simulink model "fix_Current_sync"  (R2025b)
settings: Solver=FixedStepAuto  StartTime=0.0  StopTime=20  FixedStep=0.001  RelTol=1e-3
values from neighbouring files (symbols this model uses):
  Dm = 1e-3    (= 0.001)    [motor_param.m]
  Ki_s = 0.041    [motor_param.m]
  Kp_s = 0.0014    [motor_param.m]
  Ld = 0.01    [motor_param.m]
  Lq = 0.02    [motor_param.m]
  p = 2    [motor_param.m]
  Phi = 0.1    [motor_param.m]
  Rs = 0.38    [motor_param.m]
libraries: fl_lib x50, nesl_utility x50, ee_lib x15, eeTransforms x10, slpidlib x5
(part 2 of 3)

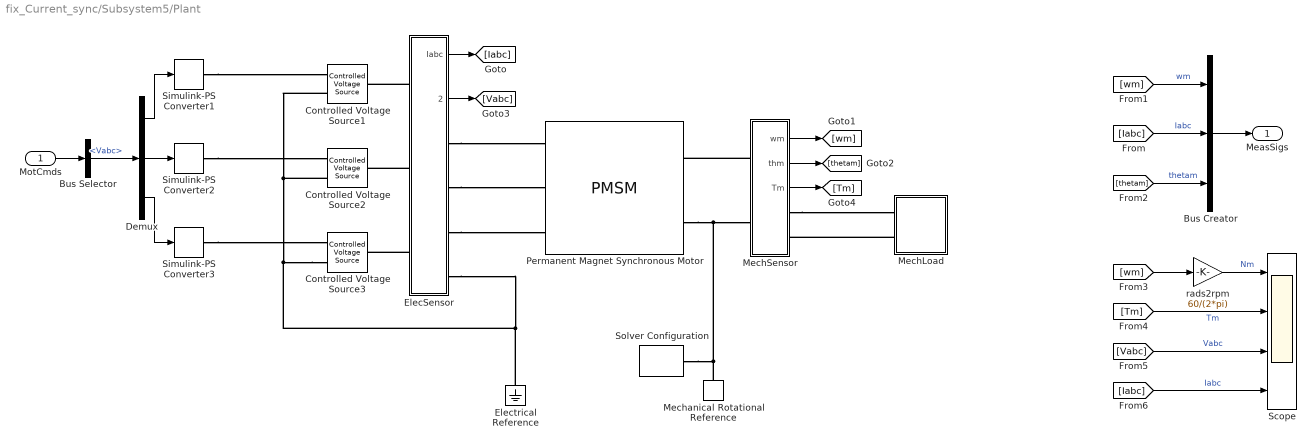
== system fix_Current_sync/Subsystem5/Plant ==
  MotCmds : Inport
  Bus Creator : BusCreator  Inputs=3
  Bus Selector : BusSelector  OutputSignals=Vabc
  Controlled Voltage Source1 : fl_lib/Electrical/Electrical Sources/Controlled Voltage Source
  Controlled Voltage Source2 : fl_lib/Electrical/Electrical Sources/Controlled Voltage Source
  Controlled Voltage Source3 : fl_lib/Electrical/Electrical Sources/Controlled Voltage Source
  Demux : Demux  Outputs=3
  ElecSensor : Subsystem
  Electrical Reference : fl_lib/Electrical/Electrical Elements/Electrical Reference
  MechLoad : Subsystem
  MechSensor : Subsystem
  Mechanical Rotational Reference : fl_lib/Mechanical/Rotational Elements/Mechanical Rotational Reference
  Permanent Magnet Synchronous Motor : ee_lib/Electromechanical/Permanent Magnet/PMSM  port_option=ee.enum.threePhasePort.expanded  winding_type=ee.enum.statorconnection.wye  machine_param=ee.enum.pmsm.parameterization.constant  nPolePairs=p  pmflux_param=1  pm_flux_linkage=Phi Wb  torque_constant=0.18 N*m/A  back_emf_constant=0.18 V/(rad/s)  stator_param=1  Ld=Ld H  Lq=Lq H  idVec=[-200, 0, 200] A  iqVec=[-200, 0, 200] A  LdMatrix=0.0002 * ones(3, 3) H  LqMatrix=0.0002 * ones(3, 3) H  PmMatrix=0.1 * ones(3, 3) Wb  ktMatrix=0.18 * ones(3, 3) N*m/A  keMatrix=0.18 * ones(3, 3) V/(rad/s)  L0=0 H  Ls=0.0002 H  Lm=-0.00002 H  Ms=0.00002 H  Rs=Rs Ohm  zero_sequence=ee.enum.park.zerosequence.exclude  axes_param=2  loss_param=ee.enum.ironloss.none  losses_oc=[0, 0, 0] W  losses_sc=[0, 0, 0] W  f_losses=60 Hz  Isc_losses=95 A  J=0 kg*m^2  lam=0 N*m/(rad/s)  i_d_specify=off  i_d_priority=None  i_d=0 A  i_d_nominal_specify=off  i_d_nominal_value=1  i_d_nominal_unit=A  i_q_specify=off  i_q_priority=None  i_q=0 A  i_q_nominal_specify=off  i_q_nominal_value=1  i_q_nominal_unit=A  torque_specify=off  torque_priority=None  torque=0 N*m  torque_nominal_specify=off  torque_nominal_value=1  torque_nominal_unit=N*m  angular_velocity_specify=on  angular_velocity_priority=High  angular_velocity=-100 rpm  angular_velocity_nominal_specify=off  angular_velocity_nominal_value=1  angular_velocity_nominal_unit=rpm  angular_position_specify=off  angular_position_priority=High  angular_position=2 rad  angular_position_nominal_specify=on  angular_position_nominal_value=10  angular_position_nominal_unit=deg  alpha=3.93e-3 1/K  alpha_flux=-0.001 1/K  Tmeas=298.15 K  stator_thermal_mass=100 J/K  rotor_thermal_mass=200 J/K  Rm_percent_rotor=90  Rd_percent_rotor=30  temperatureA_specify=off  temperatureA_priority=High  temperatureA=25 degC  temperatureA_nominal_specify=off  temperatureA_nominal_value=1  temperatureA_nominal_unit=degC  temperatureB_specify=off  temperatureB_priority=High  temperatureB=25 degC  temperatureB_nominal_specify=off  temperatureB_nominal_value=1  temperatureB_nominal_unit=degC  temperatureC_specify=off  temperatureC_priority=High  temperatureC=25 degC  temperatureC_nominal_specify=off  temperatureC_nominal_value=1  temperatureC_nominal_unit=degC  temperatureR_specify=off  temperatureR_priority=High  temperatureR=25 degC  temperatureR_nominal_specify=off  temperatureR_nominal_value=1  temperatureR_nominal_unit=degC
      settings: InternalSimscapePortConfiguration="{\"Bottom\":[],\"Left\":[{\"id\":\"a\",\"label\":\"a\",\"type\":\"foundation.electrical.electrical\"},{\"id\":\"b\",\"label\":\"b\",\"type\":\"foundation.electrical.electrical\"},{\"id\":\"c\",\"label\":\"c\",\"type\":\"foundation.electrical.electrical\"}],\"Right\":[{\"id\":\"R\",\"label\":\"R\",\"type\":\"foundation.mechanical.rotational.rotational\"},{\"id\":\"C\",\"label\":\"C\",\"type\":\"foundation.mechanical.rotational.rotational\"}],\"Top\":[]}"
  Scope : Scope  NumInputPorts=4
      settings: ActiveDisplayYMinimum=-2500.2768341970282  ActiveDisplayYMaximum=2500.1048598569782
  Simulink-PS Converter1 : nesl_utility/Simulink-PS Converter  PhysicalDomain=network_engine_domain  SubClassName=ps_input  LeftPortType=input  RightPortType=output  PseudoPeriodic=off  Frequencies=[]  NoiseDistribution=none  NoiseParameters=[]  Unit=1  AffineConversion=off  FilteringAndDerivatives=provide  SimscapeFilterOrder=1  InputFilterTimeConstant=1e-6  UdotUserProvided=0
  Simulink-PS Converter2 : nesl_utility/Simulink-PS Converter  PhysicalDomain=network_engine_domain  SubClassName=ps_input  LeftPortType=input  RightPortType=output  PseudoPeriodic=off  Frequencies=[]  NoiseDistribution=none  NoiseParameters=[]  Unit=1  AffineConversion=off  FilteringAndDerivatives=provide  SimscapeFilterOrder=1  InputFilterTimeConstant=1e-6  UdotUserProvided=0
  Simulink-PS Converter3 : nesl_utility/Simulink-PS Converter  PhysicalDomain=network_engine_domain  SubClassName=ps_input  LeftPortType=input  RightPortType=output  PseudoPeriodic=off  Frequencies=[]  NoiseDistribution=none  NoiseParameters=[]  Unit=1  AffineConversion=off  FilteringAndDerivatives=provide  SimscapeFilterOrder=1  InputFilterTimeConstant=1e-6  UdotUserProvided=0
  Solver Configuration : nesl_utility/Solver Configuration  PhysicalDomain=network_engine_domain  SubClassName=solver  LeftPortType=input  RightPortType=generic  Tones=[]  Harmonics=[]  SimulateNoise=off  Profile=off  UseLocalSampling=off  EnableSwitchedLinearOptims=on  FrequencyDomain=off  UseCCode=off  RelTol=0.001  AbsTol=1e-06  MinStep=1e-09  ToWorkspace=off  RevertToSquareIcSolve=off  NumHomotopyIterations=100  PhasorMode=off  PhasorModeNumHarmonics=1  ConsistencySolver=NEWTON_XTOL_AFTER_FTOL  IndexReductionMethod=DerivativeReplacement  DoDC=off  ResidualTolerance=1e-09  ConsistencyTolSource=GLOBAL  ConsistencyAbsTol=0.001  ConsistencyRelTol=0.001  ConsistencyTolFactor=0.001  UseLocalSolver=off  LocalSolverChoice=NE_BACKWARD_EULER_ADVANCER  ResolveIndetEquations=on  FunctionEvalNumThread=1  LocalSolverSampleTime=0.001  DoFixedCost=off  MaxNonlinIter=3  MaxModeIter=2  ComputeImpulses=off  ImpulseIterations=2  LinearAlgebra=Sparse  LinearAlgebraNumThread=0  EquationFormulation=NE_TIME_EF  DelaysMemoryBudget=1024  AutomaticFiltering=on  FilteringTimeConstant=0.001  PartitionStorageMethod=AS_NEEDED  PartitionMemoryBudget=1024  PartitionMethod=FAST  MultibodyUseLocalSolver=off  MultibodyLocalSolverChoice=ODE1  MultibodyLocalSolverSampleTime=0.001
  rads2rpm : Gain  Gain=60/(2*pi)
  MeasSigs : Outport  VectorParamsAs1DForOutWhenUnconnected=off
  wires:
  ElecSensor/1(Iabc) -> [Iabc]
  ElecSensor/2(Vabc) -> [Vabc]
  Demux/2 -> Simulink-PS Converter2/1
  Demux/1 -> Simulink-PS Converter1/1
  Demux/3 -> Simulink-PS Converter3/1
  MechSensor/1(wm) -> [wm]
  MechSensor/2(thm) -> [thetam]
  MechSensor/3(Tm) -> [Tm]
  [wm] -> Bus Creator/1  "wm"
  [Iabc] -> Bus Creator/2  "Iabc"
  [thetam] -> Bus Creator/3  "thetam"
  Bus Creator/1 -> MeasSigs/1
  MotCmds/1 -> Bus Selector/1
  Bus Selector/1 -> Demux/1  "<Vabc>"
  [wm] -> rads2rpm/1
  rads2rpm/1 -> Scope/1  "Nm"
  [Tm] -> Scope/2  "Tm"
  [Vabc] -> Scope/3  "Vabc"
  [Iabc] -> Scope/4  "Iabc"
  connections:
  Simulink-PS Converter2/RConn1 -- Controlled Voltage Source2/RConn1
  Simulink-PS Converter3/RConn1 -- Controlled Voltage Source3/RConn1
  ElecSensor/RConn3 -- Permanent Magnet Synchronous Motor/LConn3
  ElecSensor/LConn2 -- Controlled Voltage Source2/LConn1
  Controlled Voltage Source3/RConn2 -- Controlled Voltage Source1/RConn2 -- Controlled Voltage Source2/RConn2 -- ElecSensor/RConn4 -- Electrical Reference/LConn1
  ElecSensor/RConn2 -- Permanent Magnet Synchronous Motor/LConn2
  ElecSensor/RConn1 -- Permanent Magnet Synchronous Motor/LConn1
  ElecSensor/LConn3 -- Controlled Voltage Source3/LConn1
  ElecSensor/LConn1 -- Controlled Voltage Source1/LConn1
  Simulink-PS Converter1/RConn1 -- Controlled Voltage Source1/RConn1
  Permanent Magnet Synchronous Motor/RConn2 -- Solver Configuration/RConn1 -- Mechanical Rotational Reference/LConn1 -- MechSensor/LConn2
  MechSensor/RConn1 -- MechLoad/LConn1
  MechLoad/LConn2 -- MechSensor/RConn2
  MechSensor/LConn1 -- Permanent Magnet Synchronous Motor/RConn1

== system fix_Current_sync/Subsystem1/Controller/DriverPeripherals ==
  Vabc : Inport
  Break Algebraic Loop : Subsystem
  Bus Creator : BusCreator  Inputs=1
  MotCmds : Outport  VectorParamsAs1DForOutWhenUnconnected=off
  wires:
  Vabc/1 -> Break Algebraic Loop/1(In1)
  Bus Creator/1 -> MotCmds/1
  Break Algebraic Loop/1(Out1) -> Bus Creator/1  "Vabc"

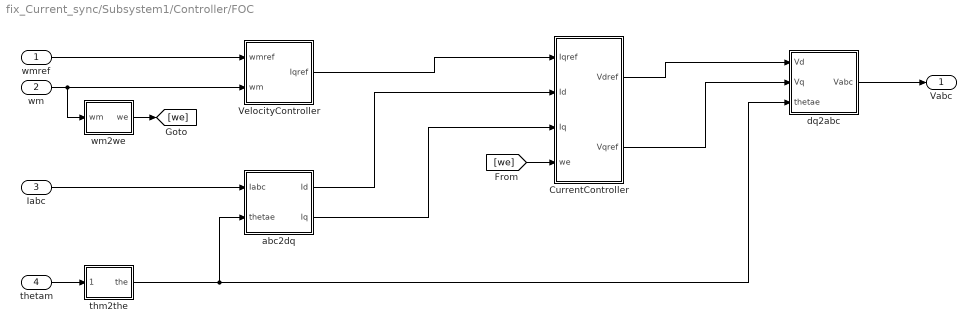
== system fix_Current_sync/Subsystem1/Controller/FOC ==
  wmref : Inport
  wm : Inport  Port=2
  Iabc : Inport  Port=3
  thetam : Inport  Port=4
  CurrentController : Subsystem
  VelocityController : Subsystem
  abc2dq : Subsystem
  dq2abc : Subsystem
  thm2the : Subsystem
  wm2we : Subsystem
  Vabc : Outport  VectorParamsAs1DForOutWhenUnconnected=off
  wires:
  abc2dq/2(Iq) -> CurrentController/3(Iq)
  wmref/1 -> VelocityController/1(wmref)
  abc2dq/1(Id) -> CurrentController/2(Id)
  Iabc/1 -> abc2dq/1(Iabc)
  CurrentController/1(Vdref) -> dq2abc/1(Vd)
  CurrentController/2(Vqref) -> dq2abc/2(Vq)
  [we] -> CurrentController/4(we)
  wm/1 -> VelocityController/2(wm), wm2we/1(wm)
  dq2abc/1(Vabc) -> Vabc/1
  VelocityController/1(Iqref) -> CurrentController/1(Iqref)
  thm2the/1(the) -> abc2dq/2(thetae), dq2abc/3(thetae)
  thetam/1 -> thm2the/1(thm)
  wm2we/1(we) -> [we]

== system fix_Current_sync/Subsystem1/Controller/SensorPeripherals ==
  MeasSigs : Inport
  Bus Selector : BusSelector  OutputSignals=wm,Iabc,thetam
  wm : Outport  VectorParamsAs1DForOutWhenUnconnected=off
  Iabc : Outport  Port=2  VectorParamsAs1DForOutWhenUnconnected=off
  thetam : Outport  Port=3  VectorParamsAs1DForOutWhenUnconnected=off
  wires:
  MeasSigs/1 -> Bus Selector/1
  Bus Selector/2 -> Iabc/1  "<Iabc>"
  Bus Selector/1 -> wm/1  "<wm>"
  Bus Selector/3 -> thetam/1  "<thetam>"

== system fix_Current_sync/Subsystem1/Controller/TestChannel ==
  TestSigs : Inport
  Bus Selector : BusSelector  OutputSignals=wmref
  wmref : Outport  VectorParamsAs1DForOutWhenUnconnected=off
  wires:
  TestSigs/1 -> Bus Selector/1
  Bus Selector/1 -> wmref/1  "<wmref>"

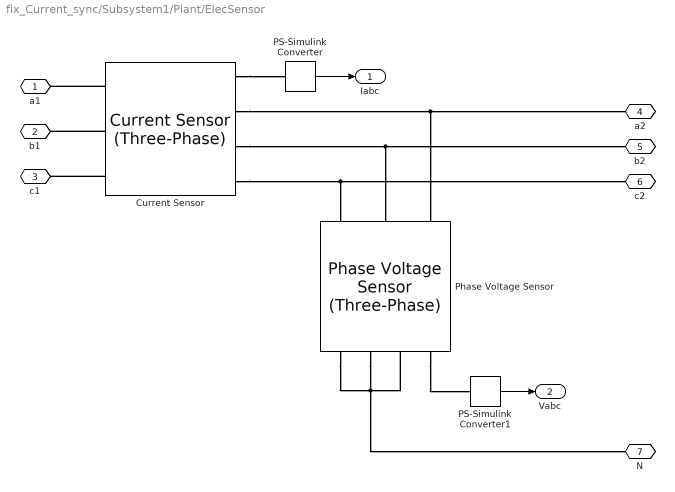
== system fix_Current_sync/Subsystem1/Plant/ElecSensor ==
  Current Sensor : ee_lib/Sensors & Transducers/Current Sensor (Three-Phase)
      settings: InternalSimscapePortConfiguration="{\"Bottom\":[],\"Left\":[{\"id\":\"a1\",\"label\":\"a1\",\"type\":\"foundation.electrical.electrical\"},{\"id\":\"b1\",\"label\":\"b1\",\"type\":\"foundation.electrical.electrical\"},{\"id\":\"c1\",\"label\":\"c1\",\"type\":\"foundation.electrical.electrical\"}],\"Right\":[{\"id\":\"I_output\",\"label\":\"I\",\"type\":\"output\"},{\"id\":\"a2\",\"label\":\"a2\",\"type\":\"foundation.electrical.electrical\"},{\"id\":\"b2\",\"label\":\"b2\",\"type\":\"foundation.electrical.electrical\"},{\"id\":\"c2\",\"label\":\"c2\",\"type\":\"foundation.electrical.electrical\"}],\"Top\":[]}"
  PS-Simulink Converter : nesl_utility/PS-Simulink Converter  PhysicalDomain=network_engine_domain  SubClassName=ps_output  LeftPortType=input  RightPortType=output  PseudoPeriodic=off  Frequencies=[]  VectorFormat=1-D array  Unit=1  AffineConversion=off
  PS-Simulink Converter1 : nesl_utility/PS-Simulink Converter  PhysicalDomain=network_engine_domain  SubClassName=ps_output  LeftPortType=input  RightPortType=output  PseudoPeriodic=off  Frequencies=[]  VectorFormat=1-D array  Unit=1  AffineConversion=off
  Phase Voltage Sensor : ee_lib/Sensors & Transducers/Phase Voltage Sensor (Three-Phase)
      settings: InternalSimscapePortConfiguration="{\"Bottom\":[],\"Left\":[{\"id\":\"a1\",\"label\":\"a1\",\"type\":\"foundation.electrical.electrical\"},{\"id\":\"b1\",\"label\":\"b1\",\"type\":\"foundation.electrical.electrical\"},{\"id\":\"c1\",\"label\":\"c1\",\"type\":\"foundation.electrical.electrical\"}],\"Right\":[{\"id\":\"V_output\",\"label\":\"V\",\"type\":\"output\"},{\"id\":\"a2\",\"label\":\"a2\",\"type\":\"foundation.electrical.electrical\"},{\"id\":\"b2\",\"label\":\"b2\",\"type\":\"foundation.electrical.electrical\"},{\"id\":\"c2\",\"label\":\"c2\",\"type\":\"foundation.electrical.electrical\"}],\"Top\":[]}"
  a1 : PMIOPort  Side=Left
  b1 : PMIOPort  Port=2  Side=Left
  c1 : PMIOPort  Port=3  Side=Left
  a2 : PMIOPort  Port=4  Side=Right
  b2 : PMIOPort  Port=5  Side=Right
  c2 : PMIOPort  Port=6  Side=Right
  N : PMIOPort  Port=7  Side=Right
  Iabc : Outport  VectorParamsAs1DForOutWhenUnconnected=off
  Vabc : Outport  Port=2  VectorParamsAs1DForOutWhenUnconnected=off
  wires:
  PS-Simulink Converter/1 -> Iabc/1
  PS-Simulink Converter1/1 -> Vabc/1
  connections:
  Current Sensor/LConn1 -- a1/RConn1
  Current Sensor/LConn2 -- b1/RConn1
  Current Sensor/LConn3 -- c1/RConn1
  Current Sensor/RConn1 -- PS-Simulink Converter/LConn1
  Phase Voltage Sensor/RConn1 -- PS-Simulink Converter1/LConn1
  Current Sensor/RConn2 -- a2/RConn1 -- Phase Voltage Sensor/LConn1
  Current Sensor/RConn3 -- b2/RConn1 -- Phase Voltage Sensor/LConn2
  Current Sensor/RConn4 -- c2/RConn1 -- Phase Voltage Sensor/LConn3
  Phase Voltage Sensor/RConn4 -- N/RConn1 -- Phase Voltage Sensor/RConn3 -- Phase Voltage Sensor/RConn2

== system fix_Current_sync/Subsystem1/Plant/MechLoad ==
  Ideal Torque Source : fl_lib/Mechanical/Mechanical Sources/Ideal Torque Source
  Inertia : fl_lib/Mechanical/Rotational Elements/Inertia  inertia=Jm kg*m^2  num_ports=foundation.enum.numPorts2.one  w_specify=on  w_priority=High  w=100 rpm  w_nominal_specify=off  w_nominal_value=1  w_nominal_unit=rad/s  t_specify=off  t_priority=None  t=0 N*m  t_nominal_specify=off  t_nominal_value=1  t_nominal_unit=N*m
  Rotational Damper : fl_lib/Mechanical/Rotational Elements/Rotational Damper  D=Dm N*m/(rad/s)  w_specify=off  w_priority=None  w=0 rad/s  w_nominal_specify=off  w_nominal_value=1  w_nominal_unit=rad/s  t_specify=off  t_priority=None  t=0 N*m  t_nominal_specify=off  t_nominal_value=1  t_nominal_unit=N*m
  Simulink-PS Converter4 : nesl_utility/Simulink-PS Converter  PhysicalDomain=network_engine_domain  SubClassName=ps_input  LeftPortType=input  RightPortType=output  PseudoPeriodic=off  Frequencies=[]  NoiseDistribution=none  NoiseParameters=[]  Unit=1  AffineConversion=off  FilteringAndDerivatives=provide  SimscapeFilterOrder=1  InputFilterTimeConstant=0.001  UdotUserProvided=0
  Step : Step  Time=0  After=0.2  SampleTime=0
  R : PMIOPort  Side=Left
  C : PMIOPort  Port=2  Side=Left
  wires:
  Step/1 -> Simulink-PS Converter4/1
  connections:
  Ideal Torque Source/RConn1 -- Simulink-PS Converter4/RConn1
  Rotational Damper/RConn1 -- Ideal Torque Source/RConn2 -- C/RConn1
  Rotational Damper/LConn1 -- Ideal Torque Source/LConn1 -- R/RConn1 -- Inertia/LConn1

== system fix_Current_sync/Subsystem1/Plant/MechSensor ==
  Ideal Rotational Motion Sensor : fl_lib/Mechanical/Mechanical Sensors/Ideal Rotational Motion Sensor  reference=foundation.enum.MeasurementReference.difference  acceleration_port=false  velocity_port=true  position_port=true  wrap_angle=simscape.enum.onoff.off  offset=0 rad
  Ideal Torque Sensor : fl_lib/Mechanical/Mechanical Sensors/Ideal Torque Sensor
  PS-Simulink Converter : nesl_utility/PS-Simulink Converter  PhysicalDomain=network_engine_domain  SubClassName=ps_output  LeftPortType=input  RightPortType=output  PseudoPeriodic=off  Frequencies=[]  VectorFormat=1-D array  Unit=1  AffineConversion=off
  PS-Simulink Converter1 : nesl_utility/PS-Simulink Converter  PhysicalDomain=network_engine_domain  SubClassName=ps_output  LeftPortType=input  RightPortType=output  PseudoPeriodic=off  Frequencies=[]  VectorFormat=1-D array  Unit=1  AffineConversion=off
  PS-Simulink Converter2 : nesl_utility/PS-Simulink Converter  PhysicalDomain=network_engine_domain  SubClassName=ps_output  LeftPortType=input  RightPortType=output  PseudoPeriodic=off  Frequencies=[]  VectorFormat=1-D array  Unit=1  AffineConversion=off
  R1 : PMIOPort  Side=Left
  C1 : PMIOPort  Port=2  Side=Left
  R2 : PMIOPort  Port=3  Side=Right
  C2 : PMIOPort  Port=4  Side=Right
  wm : Outport  VectorParamsAs1DForOutWhenUnconnected=off
  thm : Outport  Port=2  VectorParamsAs1DForOutWhenUnconnected=off
  Tm : Outport  Port=3  VectorParamsAs1DForOutWhenUnconnected=off
  wires:
  PS-Simulink Converter/1 -> thm/1
  PS-Simulink Converter1/1 -> Tm/1
  PS-Simulink Converter2/1 -> wm/1
  connections:
  Ideal Rotational Motion Sensor/RConn3 -- PS-Simulink Converter/LConn1
  Ideal Rotational Motion Sensor/RConn1 -- C2/RConn1 -- C1/RConn1
  Ideal Torque Sensor/LConn1 -- R1/RConn1
  Ideal Torque Sensor/RConn1 -- R2/RConn1 -- Ideal Rotational Motion Sensor/LConn1
  PS-Simulink Converter1/LConn1 -- Ideal Torque Sensor/RConn2
  Ideal Rotational Motion Sensor/RConn2 -- PS-Simulink Converter2/LConn1

== system fix_Current_sync/Subsystem2/Controller/DriverPeripherals ==
  Vabc : Inport
  Break Algebraic Loop : Subsystem
  Bus Creator : BusCreator  Inputs=1
  MotCmds : Outport  VectorParamsAs1DForOutWhenUnconnected=off
  wires:
  Vabc/1 -> Break Algebraic Loop/1(In1)
  Bus Creator/1 -> MotCmds/1
  Break Algebraic Loop/1(Out1) -> Bus Creator/1  "Vabc"

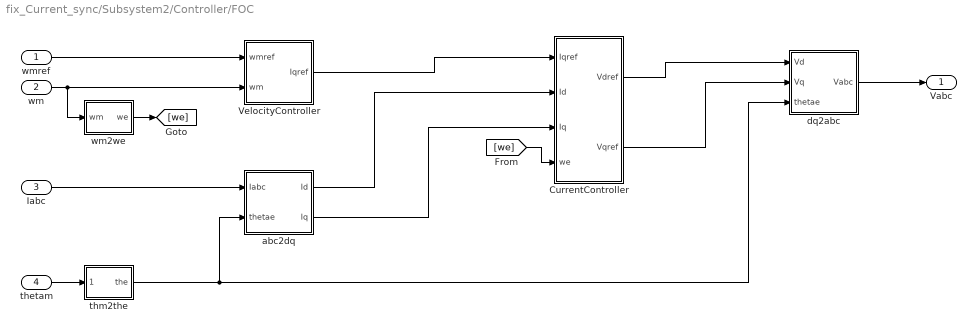
== system fix_Current_sync/Subsystem2/Controller/FOC ==
  wmref : Inport
  wm : Inport  Port=2
  Iabc : Inport  Port=3
  thetam : Inport  Port=4
  CurrentController : Subsystem
  VelocityController : Subsystem
  abc2dq : Subsystem
  dq2abc : Subsystem
  thm2the : Subsystem
  wm2we : Subsystem
  Vabc : Outport  VectorParamsAs1DForOutWhenUnconnected=off
  wires:
  abc2dq/2(Iq) -> CurrentController/3(Iq)
  wmref/1 -> VelocityController/1(wmref)
  abc2dq/1(Id) -> CurrentController/2(Id)
  Iabc/1 -> abc2dq/1(Iabc)
  CurrentController/1(Vdref) -> dq2abc/1(Vd)
  CurrentController/2(Vqref) -> dq2abc/2(Vq)
  [we] -> CurrentController/4(we)
  wm/1 -> VelocityController/2(wm), wm2we/1(wm)
  dq2abc/1(Vabc) -> Vabc/1
  VelocityController/1(Iqref) -> CurrentController/1(Iqref)
  thm2the/1(the) -> abc2dq/2(thetae), dq2abc/3(thetae)
  thetam/1 -> thm2the/1(thm)
  wm2we/1(we) -> [we]

== system fix_Current_sync/Subsystem2/Controller/SensorPeripherals ==
  MeasSigs : Inport
  Bus Selector : BusSelector  OutputSignals=wm,Iabc,thetam
  wm : Outport  VectorParamsAs1DForOutWhenUnconnected=off
  Iabc : Outport  Port=2  VectorParamsAs1DForOutWhenUnconnected=off
  thetam : Outport  Port=3  VectorParamsAs1DForOutWhenUnconnected=off
  wires:
  MeasSigs/1 -> Bus Selector/1
  Bus Selector/2 -> Iabc/1  "<Iabc>"
  Bus Selector/1 -> wm/1  "<wm>"
  Bus Selector/3 -> thetam/1  "<thetam>"

== system fix_Current_sync/Subsystem2/Controller/TestChannel ==
  TestSigs : Inport
  Bus Selector : BusSelector  OutputSignals=wmref
  wmref : Outport  VectorParamsAs1DForOutWhenUnconnected=off
  wires:
  TestSigs/1 -> Bus Selector/1
  Bus Selector/1 -> wmref/1  "<wmref>"

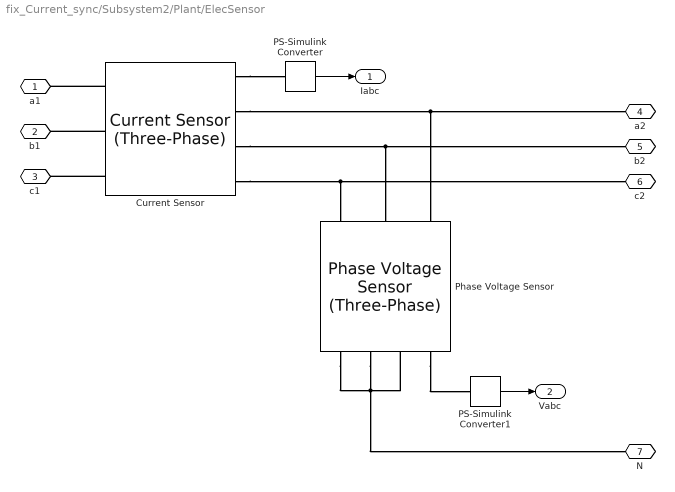
== system fix_Current_sync/Subsystem2/Plant/ElecSensor ==
  Current Sensor : ee_lib/Sensors & Transducers/Current Sensor (Three-Phase)
      settings: InternalSimscapePortConfiguration="{\"Bottom\":[],\"Left\":[{\"id\":\"a1\",\"label\":\"a1\",\"type\":\"foundation.electrical.electrical\"},{\"id\":\"b1\",\"label\":\"b1\",\"type\":\"foundation.electrical.electrical\"},{\"id\":\"c1\",\"label\":\"c1\",\"type\":\"foundation.electrical.electrical\"}],\"Right\":[{\"id\":\"I_output\",\"label\":\"I\",\"type\":\"output\"},{\"id\":\"a2\",\"label\":\"a2\",\"type\":\"foundation.electrical.electrical\"},{\"id\":\"b2\",\"label\":\"b2\",\"type\":\"foundation.electrical.electrical\"},{\"id\":\"c2\",\"label\":\"c2\",\"type\":\"foundation.electrical.electrical\"}],\"Top\":[]}"
  PS-Simulink Converter : nesl_utility/PS-Simulink Converter  PhysicalDomain=network_engine_domain  SubClassName=ps_output  LeftPortType=input  RightPortType=output  PseudoPeriodic=off  Frequencies=[]  VectorFormat=1-D array  Unit=1  AffineConversion=off
  PS-Simulink Converter1 : nesl_utility/PS-Simulink Converter  PhysicalDomain=network_engine_domain  SubClassName=ps_output  LeftPortType=input  RightPortType=output  PseudoPeriodic=off  Frequencies=[]  VectorFormat=1-D array  Unit=1  AffineConversion=off
  Phase Voltage Sensor : ee_lib/Sensors & Transducers/Phase Voltage Sensor (Three-Phase)
      settings: InternalSimscapePortConfiguration="{\"Bottom\":[],\"Left\":[{\"id\":\"a1\",\"label\":\"a1\",\"type\":\"foundation.electrical.electrical\"},{\"id\":\"b1\",\"label\":\"b1\",\"type\":\"foundation.electrical.electrical\"},{\"id\":\"c1\",\"label\":\"c1\",\"type\":\"foundation.electrical.electrical\"}],\"Right\":[{\"id\":\"V_output\",\"label\":\"V\",\"type\":\"output\"},{\"id\":\"a2\",\"label\":\"a2\",\"type\":\"foundation.electrical.electrical\"},{\"id\":\"b2\",\"label\":\"b2\",\"type\":\"foundation.electrical.electrical\"},{\"id\":\"c2\",\"label\":\"c2\",\"type\":\"foundation.electrical.electrical\"}],\"Top\":[]}"
  a1 : PMIOPort  Side=Left
  b1 : PMIOPort  Port=2  Side=Left
  c1 : PMIOPort  Port=3  Side=Left
  a2 : PMIOPort  Port=4  Side=Right
  b2 : PMIOPort  Port=5  Side=Right
  c2 : PMIOPort  Port=6  Side=Right
  N : PMIOPort  Port=7  Side=Right
  Iabc : Outport  VectorParamsAs1DForOutWhenUnconnected=off
  Vabc : Outport  Port=2  VectorParamsAs1DForOutWhenUnconnected=off
  wires:
  PS-Simulink Converter/1 -> Iabc/1
  PS-Simulink Converter1/1 -> Vabc/1
  connections:
  Current Sensor/LConn1 -- a1/RConn1
  Current Sensor/LConn2 -- b1/RConn1
  Current Sensor/LConn3 -- c1/RConn1
  Current Sensor/RConn1 -- PS-Simulink Converter/LConn1
  Phase Voltage Sensor/RConn1 -- PS-Simulink Converter1/LConn1
  Current Sensor/RConn2 -- a2/RConn1 -- Phase Voltage Sensor/LConn1
  Current Sensor/RConn3 -- b2/RConn1 -- Phase Voltage Sensor/LConn2
  Current Sensor/RConn4 -- c2/RConn1 -- Phase Voltage Sensor/LConn3
  Phase Voltage Sensor/RConn4 -- N/RConn1 -- Phase Voltage Sensor/RConn3 -- Phase Voltage Sensor/RConn2

== system fix_Current_sync/Subsystem2/Plant/MechLoad ==
  Ideal Torque Source : fl_lib/Mechanical/Mechanical Sources/Ideal Torque Source
  Inertia : fl_lib/Mechanical/Rotational Elements/Inertia  inertia=Jm kg*m^2  num_ports=foundation.enum.numPorts2.one  w_specify=on  w_priority=High  w=50 rpm  w_nominal_specify=off  w_nominal_value=1  w_nominal_unit=rad/s  t_specify=off  t_priority=None  t=0 N*m  t_nominal_specify=off  t_nominal_value=1  t_nominal_unit=N*m
  Rotational Damper : fl_lib/Mechanical/Rotational Elements/Rotational Damper  D=Dm N*m/(rad/s)  w_specify=off  w_priority=None  w=0 rad/s  w_nominal_specify=off  w_nominal_value=1  w_nominal_unit=rad/s  t_specify=off  t_priority=None  t=0 N*m  t_nominal_specify=off  t_nominal_value=1  t_nominal_unit=N*m
  Simulink-PS Converter4 : nesl_utility/Simulink-PS Converter  PhysicalDomain=network_engine_domain  SubClassName=ps_input  LeftPortType=input  RightPortType=output  PseudoPeriodic=off  Frequencies=[]  NoiseDistribution=none  NoiseParameters=[]  Unit=1  AffineConversion=off  FilteringAndDerivatives=provide  SimscapeFilterOrder=1  InputFilterTimeConstant=0.001  UdotUserProvided=0
  Step : Step  Time=0  After=0.5  SampleTime=0
  R : PMIOPort  Side=Left
  C : PMIOPort  Port=2  Side=Left
  wires:
  Step/1 -> Simulink-PS Converter4/1
  connections:
  Ideal Torque Source/RConn1 -- Simulink-PS Converter4/RConn1
  Rotational Damper/RConn1 -- Ideal Torque Source/RConn2 -- C/RConn1
  Rotational Damper/LConn1 -- Ideal Torque Source/LConn1 -- R/RConn1 -- Inertia/LConn1

== system fix_Current_sync/Subsystem2/Plant/MechSensor ==
  Ideal Rotational Motion Sensor : fl_lib/Mechanical/Mechanical Sensors/Ideal Rotational Motion Sensor  reference=foundation.enum.MeasurementReference.difference  acceleration_port=false  velocity_port=true  position_port=true  wrap_angle=simscape.enum.onoff.off  offset=0 rad
  Ideal Torque Sensor : fl_lib/Mechanical/Mechanical Sensors/Ideal Torque Sensor
  PS-Simulink Converter : nesl_utility/PS-Simulink Converter  PhysicalDomain=network_engine_domain  SubClassName=ps_output  LeftPortType=input  RightPortType=output  PseudoPeriodic=off  Frequencies=[]  VectorFormat=1-D array  Unit=1  AffineConversion=off
  PS-Simulink Converter1 : nesl_utility/PS-Simulink Converter  PhysicalDomain=network_engine_domain  SubClassName=ps_output  LeftPortType=input  RightPortType=output  PseudoPeriodic=off  Frequencies=[]  VectorFormat=1-D array  Unit=1  AffineConversion=off
  PS-Simulink Converter2 : nesl_utility/PS-Simulink Converter  PhysicalDomain=network_engine_domain  SubClassName=ps_output  LeftPortType=input  RightPortType=output  PseudoPeriodic=off  Frequencies=[]  VectorFormat=1-D array  Unit=1  AffineConversion=off
  R1 : PMIOPort  Side=Left
  C1 : PMIOPort  Port=2  Side=Left
  R2 : PMIOPort  Port=3  Side=Right
  C2 : PMIOPort  Port=4  Side=Right
  wm : Outport  VectorParamsAs1DForOutWhenUnconnected=off
  thm : Outport  Port=2  VectorParamsAs1DForOutWhenUnconnected=off
  Tm : Outport  Port=3  VectorParamsAs1DForOutWhenUnconnected=off
  wires:
  PS-Simulink Converter/1 -> thm/1
  PS-Simulink Converter1/1 -> Tm/1
  PS-Simulink Converter2/1 -> wm/1
  connections:
  Ideal Rotational Motion Sensor/RConn3 -- PS-Simulink Converter/LConn1
  Ideal Rotational Motion Sensor/RConn1 -- C2/RConn1 -- C1/RConn1
  Ideal Torque Sensor/LConn1 -- R1/RConn1
  Ideal Torque Sensor/RConn1 -- R2/RConn1 -- Ideal Rotational Motion Sensor/LConn1
  PS-Simulink Converter1/LConn1 -- Ideal Torque Sensor/RConn2
  Ideal Rotational Motion Sensor/RConn2 -- PS-Simulink Converter2/LConn1

== system fix_Current_sync/Subsystem3/Controller/DriverPeripherals ==
  Vabc : Inport
  Break Algebraic Loop : Subsystem
  Bus Creator : BusCreator  Inputs=1
  MotCmds : Outport  VectorParamsAs1DForOutWhenUnconnected=off
  wires:
  Vabc/1 -> Break Algebraic Loop/1(In1)
  Bus Creator/1 -> MotCmds/1
  Break Algebraic Loop/1(Out1) -> Bus Creator/1  "Vabc"

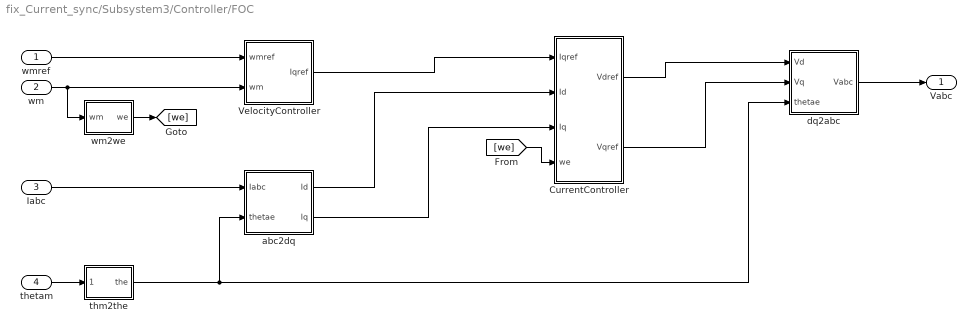
== system fix_Current_sync/Subsystem3/Controller/FOC ==
  wmref : Inport
  wm : Inport  Port=2
  Iabc : Inport  Port=3
  thetam : Inport  Port=4
  CurrentController : Subsystem
  VelocityController : Subsystem
  abc2dq : Subsystem
  dq2abc : Subsystem
  thm2the : Subsystem
  wm2we : Subsystem
  Vabc : Outport  VectorParamsAs1DForOutWhenUnconnected=off
  wires:
  abc2dq/2(Iq) -> CurrentController/3(Iq)
  wmref/1 -> VelocityController/1(wmref)
  abc2dq/1(Id) -> CurrentController/2(Id)
  Iabc/1 -> abc2dq/1(Iabc)
  CurrentController/1(Vdref) -> dq2abc/1(Vd)
  CurrentController/2(Vqref) -> dq2abc/2(Vq)
  [we] -> CurrentController/4(we)
  wm/1 -> VelocityController/2(wm), wm2we/1(wm)
  dq2abc/1(Vabc) -> Vabc/1
  VelocityController/1(Iqref) -> CurrentController/1(Iqref)
  thm2the/1(the) -> abc2dq/2(thetae), dq2abc/3(thetae)
  thetam/1 -> thm2the/1(thm)
  wm2we/1(we) -> [we]

== system fix_Current_sync/Subsystem3/Controller/SensorPeripherals ==
  MeasSigs : Inport
  Bus Selector : BusSelector  OutputSignals=wm,Iabc,thetam
  wm : Outport  VectorParamsAs1DForOutWhenUnconnected=off
  Iabc : Outport  Port=2  VectorParamsAs1DForOutWhenUnconnected=off
  thetam : Outport  Port=3  VectorParamsAs1DForOutWhenUnconnected=off
  wires:
  MeasSigs/1 -> Bus Selector/1
  Bus Selector/2 -> Iabc/1  "<Iabc>"
  Bus Selector/1 -> wm/1  "<wm>"
  Bus Selector/3 -> thetam/1  "<thetam>"

== system fix_Current_sync/Subsystem3/Controller/TestChannel ==
  TestSigs : Inport
  Bus Selector : BusSelector  OutputSignals=wmref
  wmref : Outport  VectorParamsAs1DForOutWhenUnconnected=off
  wires:
  TestSigs/1 -> Bus Selector/1
  Bus Selector/1 -> wmref/1  "<wmref>"

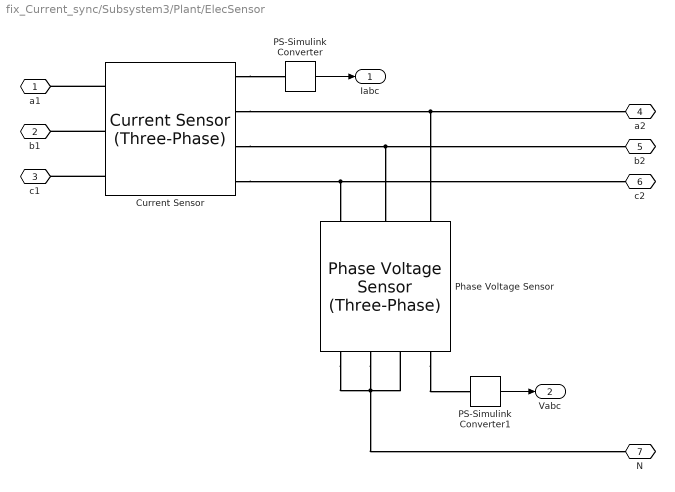
== system fix_Current_sync/Subsystem3/Plant/ElecSensor ==
  Current Sensor : ee_lib/Sensors & Transducers/Current Sensor (Three-Phase)
      settings: InternalSimscapePortConfiguration="{\"Bottom\":[],\"Left\":[{\"id\":\"a1\",\"label\":\"a1\",\"type\":\"foundation.electrical.electrical\"},{\"id\":\"b1\",\"label\":\"b1\",\"type\":\"foundation.electrical.electrical\"},{\"id\":\"c1\",\"label\":\"c1\",\"type\":\"foundation.electrical.electrical\"}],\"Right\":[{\"id\":\"I_output\",\"label\":\"I\",\"type\":\"output\"},{\"id\":\"a2\",\"label\":\"a2\",\"type\":\"foundation.electrical.electrical\"},{\"id\":\"b2\",\"label\":\"b2\",\"type\":\"foundation.electrical.electrical\"},{\"id\":\"c2\",\"label\":\"c2\",\"type\":\"foundation.electrical.electrical\"}],\"Top\":[]}"
  PS-Simulink Converter : nesl_utility/PS-Simulink Converter  PhysicalDomain=network_engine_domain  SubClassName=ps_output  LeftPortType=input  RightPortType=output  PseudoPeriodic=off  Frequencies=[]  VectorFormat=1-D array  Unit=1  AffineConversion=off
  PS-Simulink Converter1 : nesl_utility/PS-Simulink Converter  PhysicalDomain=network_engine_domain  SubClassName=ps_output  LeftPortType=input  RightPortType=output  PseudoPeriodic=off  Frequencies=[]  VectorFormat=1-D array  Unit=1  AffineConversion=off
  Phase Voltage Sensor : ee_lib/Sensors & Transducers/Phase Voltage Sensor (Three-Phase)
      settings: InternalSimscapePortConfiguration="{\"Bottom\":[],\"Left\":[{\"id\":\"a1\",\"label\":\"a1\",\"type\":\"foundation.electrical.electrical\"},{\"id\":\"b1\",\"label\":\"b1\",\"type\":\"foundation.electrical.electrical\"},{\"id\":\"c1\",\"label\":\"c1\",\"type\":\"foundation.electrical.electrical\"}],\"Right\":[{\"id\":\"V_output\",\"label\":\"V\",\"type\":\"output\"},{\"id\":\"a2\",\"label\":\"a2\",\"type\":\"foundation.electrical.electrical\"},{\"id\":\"b2\",\"label\":\"b2\",\"type\":\"foundation.electrical.electrical\"},{\"id\":\"c2\",\"label\":\"c2\",\"type\":\"foundation.electrical.electrical\"}],\"Top\":[]}"
  a1 : PMIOPort  Side=Left
  b1 : PMIOPort  Port=2  Side=Left
  c1 : PMIOPort  Port=3  Side=Left
  a2 : PMIOPort  Port=4  Side=Right
  b2 : PMIOPort  Port=5  Side=Right
  c2 : PMIOPort  Port=6  Side=Right
  N : PMIOPort  Port=7  Side=Right
  Iabc : Outport  VectorParamsAs1DForOutWhenUnconnected=off
  Vabc : Outport  Port=2  VectorParamsAs1DForOutWhenUnconnected=off
  wires:
  PS-Simulink Converter/1 -> Iabc/1
  PS-Simulink Converter1/1 -> Vabc/1
  connections:
  Current Sensor/LConn1 -- a1/RConn1
  Current Sensor/LConn2 -- b1/RConn1
  Current Sensor/LConn3 -- c1/RConn1
  Current Sensor/RConn1 -- PS-Simulink Converter/LConn1
  Phase Voltage Sensor/RConn1 -- PS-Simulink Converter1/LConn1
  Current Sensor/RConn2 -- a2/RConn1 -- Phase Voltage Sensor/LConn1
  Current Sensor/RConn3 -- b2/RConn1 -- Phase Voltage Sensor/LConn2
  Current Sensor/RConn4 -- c2/RConn1 -- Phase Voltage Sensor/LConn3
  Phase Voltage Sensor/RConn4 -- N/RConn1 -- Phase Voltage Sensor/RConn3 -- Phase Voltage Sensor/RConn2

== system fix_Current_sync/Subsystem3/Plant/MechLoad ==
  Ideal Torque Source : fl_lib/Mechanical/Mechanical Sources/Ideal Torque Source
  Inertia : fl_lib/Mechanical/Rotational Elements/Inertia  inertia=Jm kg*m^2  num_ports=foundation.enum.numPorts2.one  w_specify=on  w_priority=High  w=0 rpm  w_nominal_specify=off  w_nominal_value=1  w_nominal_unit=rad/s  t_specify=off  t_priority=None  t=0 N*m  t_nominal_specify=off  t_nominal_value=1  t_nominal_unit=N*m
  Rotational Damper : fl_lib/Mechanical/Rotational Elements/Rotational Damper  D=Dm N*m/(rad/s)  w_specify=off  w_priority=None  w=0 rad/s  w_nominal_specify=off  w_nominal_value=1  w_nominal_unit=rad/s  t_specify=off  t_priority=None  t=0 N*m  t_nominal_specify=off  t_nominal_value=1  t_nominal_unit=N*m
  Simulink-PS Converter4 : nesl_utility/Simulink-PS Converter  PhysicalDomain=network_engine_domain  SubClassName=ps_input  LeftPortType=input  RightPortType=output  PseudoPeriodic=off  Frequencies=[]  NoiseDistribution=none  NoiseParameters=[]  Unit=1  AffineConversion=off  FilteringAndDerivatives=provide  SimscapeFilterOrder=1  InputFilterTimeConstant=0.001  UdotUserProvided=0
  Step : Step  Time=0  After=-0.2  SampleTime=0
  R : PMIOPort  Side=Left
  C : PMIOPort  Port=2  Side=Left
  wires:
  Step/1 -> Simulink-PS Converter4/1
  connections:
  Ideal Torque Source/RConn1 -- Simulink-PS Converter4/RConn1
  Rotational Damper/RConn1 -- Ideal Torque Source/RConn2 -- C/RConn1
  Rotational Damper/LConn1 -- Ideal Torque Source/LConn1 -- R/RConn1 -- Inertia/LConn1

== system fix_Current_sync/Subsystem3/Plant/MechSensor ==
  Ideal Rotational Motion Sensor : fl_lib/Mechanical/Mechanical Sensors/Ideal Rotational Motion Sensor  reference=foundation.enum.MeasurementReference.difference  acceleration_port=false  velocity_port=true  position_port=true  wrap_angle=simscape.enum.onoff.off  offset=0 rad
  Ideal Torque Sensor : fl_lib/Mechanical/Mechanical Sensors/Ideal Torque Sensor
  PS-Simulink Converter : nesl_utility/PS-Simulink Converter  PhysicalDomain=network_engine_domain  SubClassName=ps_output  LeftPortType=input  RightPortType=output  PseudoPeriodic=off  Frequencies=[]  VectorFormat=1-D array  Unit=1  AffineConversion=off
  PS-Simulink Converter1 : nesl_utility/PS-Simulink Converter  PhysicalDomain=network_engine_domain  SubClassName=ps_output  LeftPortType=input  RightPortType=output  PseudoPeriodic=off  Frequencies=[]  VectorFormat=1-D array  Unit=1  AffineConversion=off
  PS-Simulink Converter2 : nesl_utility/PS-Simulink Converter  PhysicalDomain=network_engine_domain  SubClassName=ps_output  LeftPortType=input  RightPortType=output  PseudoPeriodic=off  Frequencies=[]  VectorFormat=1-D array  Unit=1  AffineConversion=off
  R1 : PMIOPort  Side=Left
  C1 : PMIOPort  Port=2  Side=Left
  R2 : PMIOPort  Port=3  Side=Right
  C2 : PMIOPort  Port=4  Side=Right
  wm : Outport  VectorParamsAs1DForOutWhenUnconnected=off
  thm : Outport  Port=2  VectorParamsAs1DForOutWhenUnconnected=off
  Tm : Outport  Port=3  VectorParamsAs1DForOutWhenUnconnected=off
  wires:
  PS-Simulink Converter/1 -> thm/1
  PS-Simulink Converter1/1 -> Tm/1
  PS-Simulink Converter2/1 -> wm/1
  connections:
  Ideal Rotational Motion Sensor/RConn3 -- PS-Simulink Converter/LConn1
  Ideal Rotational Motion Sensor/RConn1 -- C2/RConn1 -- C1/RConn1
  Ideal Torque Sensor/LConn1 -- R1/RConn1
  Ideal Torque Sensor/RConn1 -- R2/RConn1 -- Ideal Rotational Motion Sensor/LConn1
  PS-Simulink Converter1/LConn1 -- Ideal Torque Sensor/RConn2
  Ideal Rotational Motion Sensor/RConn2 -- PS-Simulink Converter2/LConn1

== system fix_Current_sync/Subsystem4/Controller/DriverPeripherals ==
  Vabc : Inport
  Break Algebraic Loop : Subsystem
  Bus Creator : BusCreator  Inputs=1
  MotCmds : Outport  VectorParamsAs1DForOutWhenUnconnected=off
  wires:
  Vabc/1 -> Break Algebraic Loop/1(In1)
  Bus Creator/1 -> MotCmds/1
  Break Algebraic Loop/1(Out1) -> Bus Creator/1  "Vabc"

== system fix_Current_sync/Subsystem4/Controller/FOC ==
  wmref : Inport
  wm : Inport  Port=2
  Iabc : Inport  Port=3
  thetam : Inport  Port=4
  CurrentController : Subsystem
  VelocityController : Subsystem
  abc2dq : Subsystem
  dq2abc : Subsystem
  thm2the : Subsystem
  wm2we : Subsystem
  Vabc : Outport  VectorParamsAs1DForOutWhenUnconnected=off
  wires:
  abc2dq/2(Iq) -> CurrentController/3(Iq)
  wmref/1 -> VelocityController/1(wmref)
  abc2dq/1(Id) -> CurrentController/2(Id)
  Iabc/1 -> abc2dq/1(Iabc)
  CurrentController/1(Vdref) -> dq2abc/1(Vd)
  CurrentController/2(Vqref) -> dq2abc/2(Vq)
  [we] -> CurrentController/4(we)
  wm/1 -> VelocityController/2(wm), wm2we/1(wm)
  dq2abc/1(Vabc) -> Vabc/1
  VelocityController/1(Iqref) -> CurrentController/1(Iqref)
  thm2the/1(the) -> abc2dq/2(thetae), dq2abc/3(thetae)
  thetam/1 -> thm2the/1(thm)
  wm2we/1(we) -> [we]

== system fix_Current_sync/Subsystem4/Controller/SensorPeripherals ==
  MeasSigs : Inport
  Bus Selector : BusSelector  OutputSignals=wm,Iabc,thetam
  wm : Outport  VectorParamsAs1DForOutWhenUnconnected=off
  Iabc : Outport  Port=2  VectorParamsAs1DForOutWhenUnconnected=off
  thetam : Outport  Port=3  VectorParamsAs1DForOutWhenUnconnected=off
  wires:
  MeasSigs/1 -> Bus Selector/1
  Bus Selector/2 -> Iabc/1  "<Iabc>"
  Bus Selector/1 -> wm/1  "<wm>"
  Bus Selector/3 -> thetam/1  "<thetam>"

== system fix_Current_sync/Subsystem4/Controller/TestChannel ==
  TestSigs : Inport
  Bus Selector : BusSelector  OutputSignals=wmref
  wmref : Outport  VectorParamsAs1DForOutWhenUnconnected=off
  wires:
  TestSigs/1 -> Bus Selector/1
  Bus Selector/1 -> wmref/1  "<wmref>"

== system fix_Current_sync/Subsystem4/Plant/ElecSensor ==
  Current Sensor : ee_lib/Sensors & Transducers/Current Sensor (Three-Phase)
      settings: InternalSimscapePortConfiguration="{\"Bottom\":[],\"Left\":[{\"id\":\"a1\",\"label\":\"a1\",\"type\":\"foundation.electrical.electrical\"},{\"id\":\"b1\",\"label\":\"b1\",\"type\":\"foundation.electrical.electrical\"},{\"id\":\"c1\",\"label\":\"c1\",\"type\":\"foundation.electrical.electrical\"}],\"Right\":[{\"id\":\"I_output\",\"label\":\"I\",\"type\":\"output\"},{\"id\":\"a2\",\"label\":\"a2\",\"type\":\"foundation.electrical.electrical\"},{\"id\":\"b2\",\"label\":\"b2\",\"type\":\"foundation.electrical.electrical\"},{\"id\":\"c2\",\"label\":\"c2\",\"type\":\"foundation.electrical.electrical\"}],\"Top\":[]}"
  PS-Simulink Converter : nesl_utility/PS-Simulink Converter  PhysicalDomain=network_engine_domain  SubClassName=ps_output  LeftPortType=input  RightPortType=output  PseudoPeriodic=off  Frequencies=[]  VectorFormat=1-D array  Unit=1  AffineConversion=off
  PS-Simulink Converter1 : nesl_utility/PS-Simulink Converter  PhysicalDomain=network_engine_domain  SubClassName=ps_output  LeftPortType=input  RightPortType=output  PseudoPeriodic=off  Frequencies=[]  VectorFormat=1-D array  Unit=1  AffineConversion=off
  Phase Voltage Sensor : ee_lib/Sensors & Transducers/Phase Voltage Sensor (Three-Phase)
      settings: InternalSimscapePortConfiguration="{\"Bottom\":[],\"Left\":[{\"id\":\"a1\",\"label\":\"a1\",\"type\":\"foundation.electrical.electrical\"},{\"id\":\"b1\",\"label\":\"b1\",\"type\":\"foundation.electrical.electrical\"},{\"id\":\"c1\",\"label\":\"c1\",\"type\":\"foundation.electrical.electrical\"}],\"Right\":[{\"id\":\"V_output\",\"label\":\"V\",\"type\":\"output\"},{\"id\":\"a2\",\"label\":\"a2\",\"type\":\"foundation.electrical.electrical\"},{\"id\":\"b2\",\"label\":\"b2\",\"type\":\"foundation.electrical.electrical\"},{\"id\":\"c2\",\"label\":\"c2\",\"type\":\"foundation.electrical.electrical\"}],\"Top\":[]}"
  a1 : PMIOPort  Side=Left
  b1 : PMIOPort  Port=2  Side=Left
  c1 : PMIOPort  Port=3  Side=Left
  a2 : PMIOPort  Port=4  Side=Right
  b2 : PMIOPort  Port=5  Side=Right
  c2 : PMIOPort  Port=6  Side=Right
  N : PMIOPort  Port=7  Side=Right
  Iabc : Outport  VectorParamsAs1DForOutWhenUnconnected=off
  Vabc : Outport  Port=2  VectorParamsAs1DForOutWhenUnconnected=off
  wires:
  PS-Simulink Converter/1 -> Iabc/1
  PS-Simulink Converter1/1 -> Vabc/1
  connections:
  Current Sensor/LConn1 -- a1/RConn1
  Current Sensor/LConn2 -- b1/RConn1
  Current Sensor/LConn3 -- c1/RConn1
  Current Sensor/RConn1 -- PS-Simulink Converter/LConn1
  Phase Voltage Sensor/RConn1 -- PS-Simulink Converter1/LConn1
  Current Sensor/RConn2 -- a2/RConn1 -- Phase Voltage Sensor/LConn1
  Current Sensor/RConn3 -- b2/RConn1 -- Phase Voltage Sensor/LConn2
  Current Sensor/RConn4 -- c2/RConn1 -- Phase Voltage Sensor/LConn3
  Phase Voltage Sensor/RConn4 -- N/RConn1 -- Phase Voltage Sensor/RConn3 -- Phase Voltage Sensor/RConn2

== system fix_Current_sync/Subsystem4/Plant/MechLoad ==
  Ideal Torque Source : fl_lib/Mechanical/Mechanical Sources/Ideal Torque Source
  Inertia : fl_lib/Mechanical/Rotational Elements/Inertia  inertia=Jm kg*m^2  num_ports=foundation.enum.numPorts2.one  w_specify=on  w_priority=High  w=-50 rpm  w_nominal_specify=off  w_nominal_value=1  w_nominal_unit=rad/s  t_specify=off  t_priority=None  t=0 N*m  t_nominal_specify=off  t_nominal_value=1  t_nominal_unit=N*m
  Rotational Damper : fl_lib/Mechanical/Rotational Elements/Rotational Damper  D=Dm N*m/(rad/s)  w_specify=off  w_priority=None  w=0 rad/s  w_nominal_specify=off  w_nominal_value=1  w_nominal_unit=rad/s  t_specify=off  t_priority=None  t=0 N*m  t_nominal_specify=off  t_nominal_value=1  t_nominal_unit=N*m
  Simulink-PS Converter4 : nesl_utility/Simulink-PS Converter  PhysicalDomain=network_engine_domain  SubClassName=ps_input  LeftPortType=input  RightPortType=output  PseudoPeriodic=off  Frequencies=[]  NoiseDistribution=none  NoiseParameters=[]  Unit=1  AffineConversion=off  FilteringAndDerivatives=provide  SimscapeFilterOrder=1  InputFilterTimeConstant=0.001  UdotUserProvided=0
  Step : Step  Time=0  After=0  SampleTime=0
  R : PMIOPort  Side=Left
  C : PMIOPort  Port=2  Side=Left
  wires:
  Step/1 -> Simulink-PS Converter4/1
  connections:
  Ideal Torque Source/RConn1 -- Simulink-PS Converter4/RConn1
  Rotational Damper/RConn1 -- Ideal Torque Source/RConn2 -- C/RConn1
  Rotational Damper/LConn1 -- Ideal Torque Source/LConn1 -- R/RConn1 -- Inertia/LConn1

== system fix_Current_sync/Subsystem4/Plant/MechSensor ==
  Ideal Rotational Motion Sensor : fl_lib/Mechanical/Mechanical Sensors/Ideal Rotational Motion Sensor  reference=foundation.enum.MeasurementReference.difference  acceleration_port=false  velocity_port=true  position_port=true  wrap_angle=simscape.enum.onoff.off  offset=0 rad
  Ideal Torque Sensor : fl_lib/Mechanical/Mechanical Sensors/Ideal Torque Sensor
  PS-Simulink Converter : nesl_utility/PS-Simulink Converter  PhysicalDomain=network_engine_domain  SubClassName=ps_output  LeftPortType=input  RightPortType=output  PseudoPeriodic=off  Frequencies=[]  VectorFormat=1-D array  Unit=1  AffineConversion=off
  PS-Simulink Converter1 : nesl_utility/PS-Simulink Converter  PhysicalDomain=network_engine_domain  SubClassName=ps_output  LeftPortType=input  RightPortType=output  PseudoPeriodic=off  Frequencies=[]  VectorFormat=1-D array  Unit=1  AffineConversion=off
  PS-Simulink Converter2 : nesl_utility/PS-Simulink Converter  PhysicalDomain=network_engine_domain  SubClassName=ps_output  LeftPortType=input  RightPortType=output  PseudoPeriodic=off  Frequencies=[]  VectorFormat=1-D array  Unit=1  AffineConversion=off
  R1 : PMIOPort  Side=Left
  C1 : PMIOPort  Port=2  Side=Left
  R2 : PMIOPort  Port=3  Side=Right
  C2 : PMIOPort  Port=4  Side=Right
  wm : Outport  VectorParamsAs1DForOutWhenUnconnected=off
  thm : Outport  Port=2  VectorParamsAs1DForOutWhenUnconnected=off
  Tm : Outport  Port=3  VectorParamsAs1DForOutWhenUnconnected=off
  wires:
  PS-Simulink Converter/1 -> thm/1
  PS-Simulink Converter1/1 -> Tm/1
  PS-Simulink Converter2/1 -> wm/1
  connections:
  Ideal Rotational Motion Sensor/RConn3 -- PS-Simulink Converter/LConn1
  Ideal Rotational Motion Sensor/RConn1 -- C2/RConn1 -- C1/RConn1
  Ideal Torque Sensor/LConn1 -- R1/RConn1
  Ideal Torque Sensor/RConn1 -- R2/RConn1 -- Ideal Rotational Motion Sensor/LConn1
  PS-Simulink Converter1/LConn1 -- Ideal Torque Sensor/RConn2
  Ideal Rotational Motion Sensor/RConn2 -- PS-Simulink Converter2/LConn1

== system fix_Current_sync/Subsystem5/Controller/DriverPeripherals ==
  Vabc : Inport
  Break Algebraic Loop : Subsystem
  Bus Creator : BusCreator  Inputs=1
  MotCmds : Outport  VectorParamsAs1DForOutWhenUnconnected=off
  wires:
  Vabc/1 -> Break Algebraic Loop/1(In1)
  Bus Creator/1 -> MotCmds/1
  Break Algebraic Loop/1(Out1) -> Bus Creator/1  "Vabc"

== system fix_Current_sync/Subsystem5/Controller/FOC ==
  wmref : Inport
  wm : Inport  Port=2
  Iabc : Inport  Port=3
  thetam : Inport  Port=4
  CurrentController : Subsystem
  VelocityController : Subsystem
  abc2dq : Subsystem
  dq2abc : Subsystem
  thm2the : Subsystem
  wm2we : Subsystem
  Vabc : Outport  VectorParamsAs1DForOutWhenUnconnected=off
  wires:
  abc2dq/2(Iq) -> CurrentController/3(Iq)
  wmref/1 -> VelocityController/1(wmref)
  abc2dq/1(Id) -> CurrentController/2(Id)
  Iabc/1 -> abc2dq/1(Iabc)
  CurrentController/1(Vdref) -> dq2abc/1(Vd)
  CurrentController/2(Vqref) -> dq2abc/2(Vq)
  [we] -> CurrentController/4(we)
  wm/1 -> VelocityController/2(wm), wm2we/1(wm)
  dq2abc/1(Vabc) -> Vabc/1
  VelocityController/1(Iqref) -> CurrentController/1(Iqref)
  thm2the/1(the) -> abc2dq/2(thetae), dq2abc/3(thetae)
  thetam/1 -> thm2the/1(thm)
  wm2we/1(we) -> [we]

== system fix_Current_sync/Subsystem5/Controller/SensorPeripherals ==
  MeasSigs : Inport
  Bus Selector : BusSelector  OutputSignals=wm,Iabc,thetam
  wm : Outport  VectorParamsAs1DForOutWhenUnconnected=off
  Iabc : Outport  Port=2  VectorParamsAs1DForOutWhenUnconnected=off
  thetam : Outport  Port=3  VectorParamsAs1DForOutWhenUnconnected=off
  wires:
  MeasSigs/1 -> Bus Selector/1
  Bus Selector/2 -> Iabc/1  "<Iabc>"
  Bus Selector/1 -> wm/1  "<wm>"
  Bus Selector/3 -> thetam/1  "<thetam>"

== system fix_Current_sync/Subsystem5/Controller/TestChannel ==
  TestSigs : Inport
  Bus Selector : BusSelector  OutputSignals=wmref
  wmref : Outport  VectorParamsAs1DForOutWhenUnconnected=off
  wires:
  TestSigs/1 -> Bus Selector/1
  Bus Selector/1 -> wmref/1  "<wmref>"

== system fix_Current_sync/Subsystem5/Plant/ElecSensor ==
  Current Sensor : ee_lib/Sensors & Transducers/Current Sensor (Three-Phase)
      settings: InternalSimscapePortConfiguration="{\"Bottom\":[],\"Left\":[{\"id\":\"a1\",\"label\":\"a1\",\"type\":\"foundation.electrical.electrical\"},{\"id\":\"b1\",\"label\":\"b1\",\"type\":\"foundation.electrical.electrical\"},{\"id\":\"c1\",\"label\":\"c1\",\"type\":\"foundation.electrical.electrical\"}],\"Right\":[{\"id\":\"I_output\",\"label\":\"I\",\"type\":\"output\"},{\"id\":\"a2\",\"label\":\"a2\",\"type\":\"foundation.electrical.electrical\"},{\"id\":\"b2\",\"label\":\"b2\",\"type\":\"foundation.electrical.electrical\"},{\"id\":\"c2\",\"label\":\"c2\",\"type\":\"foundation.electrical.electrical\"}],\"Top\":[]}"
  PS-Simulink Converter : nesl_utility/PS-Simulink Converter  PhysicalDomain=network_engine_domain  SubClassName=ps_output  LeftPortType=input  RightPortType=output  PseudoPeriodic=off  Frequencies=[]  VectorFormat=1-D array  Unit=1  AffineConversion=off
  PS-Simulink Converter1 : nesl_utility/PS-Simulink Converter  PhysicalDomain=network_engine_domain  SubClassName=ps_output  LeftPortType=input  RightPortType=output  PseudoPeriodic=off  Frequencies=[]  VectorFormat=1-D array  Unit=1  AffineConversion=off
  Phase Voltage Sensor : ee_lib/Sensors & Transducers/Phase Voltage Sensor (Three-Phase)
      settings: InternalSimscapePortConfiguration="{\"Bottom\":[],\"Left\":[{\"id\":\"a1\",\"label\":\"a1\",\"type\":\"foundation.electrical.electrical\"},{\"id\":\"b1\",\"label\":\"b1\",\"type\":\"foundation.electrical.electrical\"},{\"id\":\"c1\",\"label\":\"c1\",\"type\":\"foundation.electrical.electrical\"}],\"Right\":[{\"id\":\"V_output\",\"label\":\"V\",\"type\":\"output\"},{\"id\":\"a2\",\"label\":\"a2\",\"type\":\"foundation.electrical.electrical\"},{\"id\":\"b2\",\"label\":\"b2\",\"type\":\"foundation.electrical.electrical\"},{\"id\":\"c2\",\"label\":\"c2\",\"type\":\"foundation.electrical.electrical\"}],\"Top\":[]}"
  a1 : PMIOPort  Side=Left
  b1 : PMIOPort  Port=2  Side=Left
  c1 : PMIOPort  Port=3  Side=Left
  a2 : PMIOPort  Port=4  Side=Right
  b2 : PMIOPort  Port=5  Side=Right
  c2 : PMIOPort  Port=6  Side=Right
  N : PMIOPort  Port=7  Side=Right
  Iabc : Outport  VectorParamsAs1DForOutWhenUnconnected=off
  Vabc : Outport  Port=2  VectorParamsAs1DForOutWhenUnconnected=off
  wires:
  PS-Simulink Converter/1 -> Iabc/1
  PS-Simulink Converter1/1 -> Vabc/1
  connections:
  Current Sensor/LConn1 -- a1/RConn1
  Current Sensor/LConn2 -- b1/RConn1
  Current Sensor/LConn3 -- c1/RConn1
  Current Sensor/RConn1 -- PS-Simulink Converter/LConn1
  Phase Voltage Sensor/RConn1 -- PS-Simulink Converter1/LConn1
  Current Sensor/RConn2 -- a2/RConn1 -- Phase Voltage Sensor/LConn1
  Current Sensor/RConn3 -- b2/RConn1 -- Phase Voltage Sensor/LConn2
  Current Sensor/RConn4 -- c2/RConn1 -- Phase Voltage Sensor/LConn3
  Phase Voltage Sensor/RConn4 -- N/RConn1 -- Phase Voltage Sensor/RConn3 -- Phase Voltage Sensor/RConn2

== system fix_Current_sync/Subsystem5/Plant/MechLoad ==
  Ideal Torque Source : fl_lib/Mechanical/Mechanical Sources/Ideal Torque Source
  Inertia : fl_lib/Mechanical/Rotational Elements/Inertia  inertia=Jm kg*m^2  num_ports=foundation.enum.numPorts2.one  w_specify=on  w_priority=High  w=-100 rpm  w_nominal_specify=off  w_nominal_value=1  w_nominal_unit=rad/s  t_specify=off  t_priority=None  t=0 N*m  t_nominal_specify=off  t_nominal_value=1  t_nominal_unit=N*m
  Rotational Damper : fl_lib/Mechanical/Rotational Elements/Rotational Damper  D=Dm N*m/(rad/s)  w_specify=off  w_priority=None  w=0 rad/s  w_nominal_specify=off  w_nominal_value=1  w_nominal_unit=rad/s  t_specify=off  t_priority=None  t=0 N*m  t_nominal_specify=off  t_nominal_value=1  t_nominal_unit=N*m
  Simulink-PS Converter4 : nesl_utility/Simulink-PS Converter  PhysicalDomain=network_engine_domain  SubClassName=ps_input  LeftPortType=input  RightPortType=output  PseudoPeriodic=off  Frequencies=[]  NoiseDistribution=none  NoiseParameters=[]  Unit=1  AffineConversion=off  FilteringAndDerivatives=provide  SimscapeFilterOrder=1  InputFilterTimeConstant=0.001  UdotUserProvided=0
  Step : Step  Time=0  After=-0.5  SampleTime=0
  R : PMIOPort  Side=Left
  C : PMIOPort  Port=2  Side=Left
  wires:
  Step/1 -> Simulink-PS Converter4/1
  connections:
  Ideal Torque Source/RConn1 -- Simulink-PS Converter4/RConn1
  Rotational Damper/RConn1 -- Ideal Torque Source/RConn2 -- C/RConn1
  Rotational Damper/LConn1 -- Ideal Torque Source/LConn1 -- R/RConn1 -- Inertia/LConn1
